simulink model "Regenerative_Braking_Trapezoidal_Control"  (R2023a)
settings: Solver=VariableStepAuto  StartTime=0.0  StopTime=10  RelTol=1e-3
undefined symbols (not defined in the file): Ion, Lithium
libraries: simulink x7, slpidlib x2, spsMeanLib x2, spsPermanentMagnetSynchronousMachineLib x1, spsBatteryLib x1, spsCurrentMeasurementLib x1, spsGroundLib x1, eePwmGenerator x1, spsUniversalBridgeLib x1, spsVoltageMeasurementLib x1, spspowerguiLib x1
settings Model: Creator=Kalyani  LastModifiedBy=hanna
settings DataIOCC: ReturnWorkspaceOutputs=off
settings RTWCC: GPUComputeCapability=5.0
settings ConfigComp: CovBoundaryAbsTol=1.0e-5

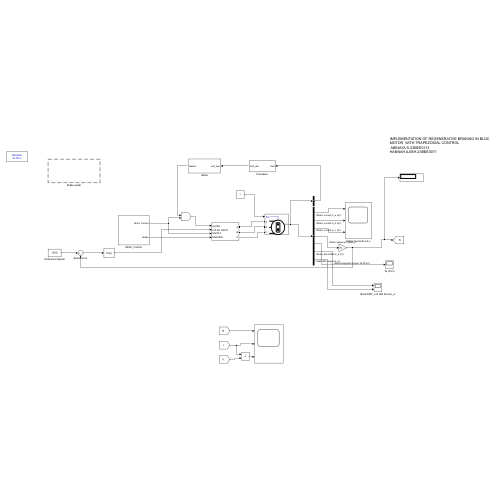
[thumbnail: Simulink's stored preview of the top-level diagram]
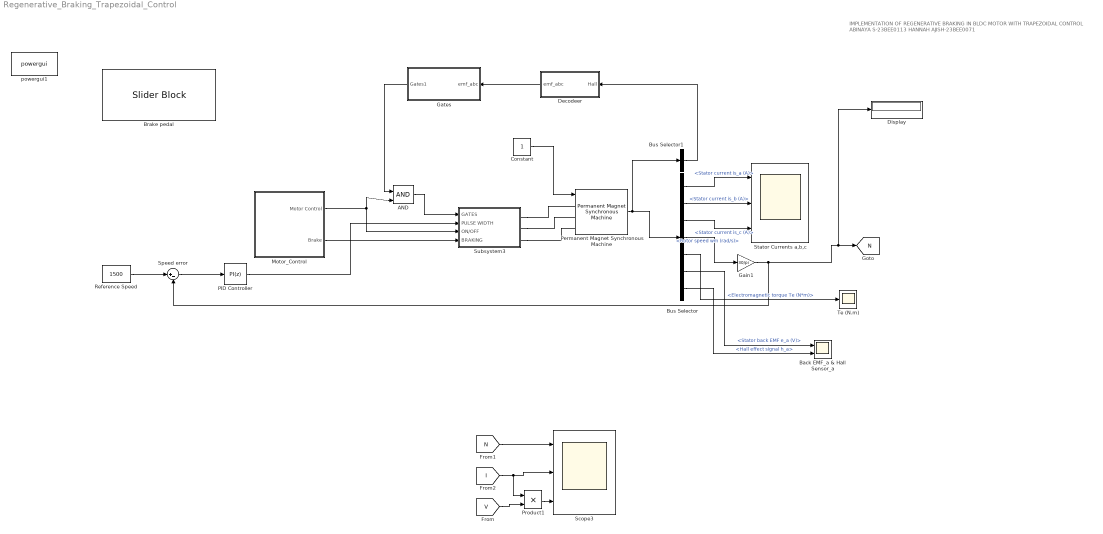
== system Regenerative_Braking_Trapezoidal_Control ==
  note: IMPLEMENTATION OF REGENERATIVE BRAKING IN BLDC MOTOR WITH TRAPEZOIDAL CONTROL
      | ABINAYA S-23BEE0113
      | HANNAH AJISH-23BEE0071
  AND : Logic  IconShape=distinctive  AllPortsSameDT=off  OutDataTypeStr=boolean
  Back EMF_a & Hall Sensor_a : Scope  NumInputPorts=2
  Brake pedal : SliderBlock  ScaleMax=0.949999
  Bus Selector : BusSelector  OutputSignals=Stator current is_a (A),Stator current is_b (A),Stator current is_c (A),Rotor speed wm (rad/s),Electromagnetic torque Te (N*m),Stator back EMF e_a (V),Hall effect signal h_a
  Bus Selector1 : BusSelector  OutputSignals=Hall effect signal h_a,Hall effect signal h_b,Hall effect signal h_c  OutputAsBus=on
  Constant : Constant
  Decodeer : Subsystem
  Display : Display
  Gain1 : Gain  Gain=30/pi
  Gates : Subsystem
  Motor_Control : Subsystem
  PID Controller : slpidlib/PID Controller  Controller=PI  Form=Parallel  TimeDomain=Discrete-time  UseExternalTs=off  SampleTime=-1  IntegratorMethod=Forward Euler  FilterMethod=Forward Euler  ControllerParametersSource=internal  P=0.014  I=0.2288  UseKiTs=off  D=0  N=100  UseFilter=on  TunerSelectOption=Transfer Function Based (PID Tuner App)  InitialConditionSource=internal  InitialConditionForIntegrator=0  InitialConditionForFilter=0  DifferentiatorICPrevScaledInput=0  ExternalReset=none  TrackingMode=off  Kt=1  LimitOutput=off  SatLimitsSource=internal  UpperSaturationLimit=inf  LowerSaturationLimit=-inf  LinearizeAsGain=on  AntiWindupMode=none  Kb=1  LimitIntegrator=off  UpperIntegratorSaturationLimit=inf  LowerIntegratorSaturationLimit=-inf  POutMin=[]  POutMax=[]  IOutMin=[]  IOutMax=[]  DOutMin=[]  DOutMax=[]  NOutMin=[]  NOutMax=[]  SumOutMin=[]  SumOutMax=[]  SaturationOutMin=[]  SaturationOutMax=[]  PParamMin=[]  PParamMax=[]  IParamMin=[]  IParamMax=[]  DParamMin=[]  DParamMax=[]  NParamMin=[]  NParamMax=[]  KbParamMin=[]  KbParamMax=[]  KtParamMin=[]  KtParamMax=[]  KbOutMin=[]  KbOutMax=[]  KtOutMin=[]  KtOutMax=[]  IntegratorOutMin=[]  IntegratorOutMax=[]  FilterOutMin=[]  FilterOutMax=[]  SumI1OutMin=[]  SumI1OutMax=[]  SumI2OutMin=[]  SumI2OutMax=[]  SumI3OutMin=[]  SumI3OutMax=[]  SumI4OutMin=[]  SumI4OutMax=[]  SumDOutMin=[]  SumDOutMax=[]  DifferentiatorOutMin=[]  DifferentiatorOutMax=[]  FilterDiffOutCoefMin=[]  FilterDiffOutCoefMax=[]  ReciprocalOutMin=[]  ReciprocalOutMax=[]  SumDenOutMin=[]  SumDenOutMax=[]  SumNumOutMin=[]  SumNumOutMax=[]  DivideOutMin=[]  DivideOutMax=[]  UdiffTsProdOutMin=[]  UdiffTsProdOutMax=[]  NTsProdOutMin=[]  NTsProdOutMax=[]  UintegralTsProdOutMin=[]  UintegralTsProdOutMax=[]  UngainTsProdOutMin=[]  UngainTsProdOutMax=[]  ClampingZeroOutDataTypeStr=Inherit: Inherit via back propagation  ClampingZeroOutMin=[]  ClampingZeroOutMax=[]  FilterDenConstantOutDataTypeStr=Inherit: Inherit via back propagation  FilterDenConstantOutMin=[]  FilterDenConstantOutMax=[]  PCopyOutDataTypeStr=Inherit: Inherit via back propagation  PCopyOutMin=[]  PCopyOutMax=[]  NCopyOutDataTypeStr=Inherit: Inherit via back propagation  NCopyOutMin=[]  NCopyOutMax=[]  IntegratorContinuousStateAttributes=''  IntegratorStateMustResolveToSignalObject=off  IntegratorRTWStateStorageClass=Auto  FilterContinuousStateAttributes=''  FilterStateMustResolveToSignalObject=off  FilterRTWStateStorageClass=Auto  ParallelPVariant=InternalParameters  IdealPVariant=Disabled  IVariant=InternalParameters  DVariant=Disabled  IntegratorVariant=Discrete  SatVariant=Disabled  AWVariant=Passthrough  PCopyVariant=Disabled  TRVariant=Disabled  FdbkBlocksVariant=Forward  IdealPFdbkVariant=Disabled  SatFdbkVariant=Disabled  DerivativeFilterVariant=Disabled  NVariant=Disabled  NCopyVariant=Disabled_SignalSpec  FilterICVariant=Disabled  IntegratorICVariant=InternalICs  ExternalResetVariant=Disabled  TRSumVariant=Passthrough  SumFdbkVariant=Disabled  SumVariant=Sum_PI  TsampFilterVariant=InternalTs  TsampNgainVariant=Passthrough  TsampIntegralVariant=Disabled_SignalSpec  ExternalSaturationOutDataTypeStr=Inherit: Same as second input
  Permanent Magnet Synchronous Machine : spsPermanentMagnetSynchronousMachineLib/Permanent Magnet Synchronous Machine  NbPhases=3  FluxDistribution=Trapezoidal  RotorType=Round  MechanicalLoad=Torque Tm  PresetModel=No  ShowDetailedParameters=on  MeasurementBus=off  Resistance=0.0095  Inductance=0.0144e-3  dqInductances=[8.5e-3,8.5e-3]  La=0.000395  MachineConstant=Torque Constant (N.m / A_peak)  Flux=0.030794  VoltageCst=51.5954  TorqueCst=0.4927  Flat=120  Mechanical=[0.00019, 1e-6, 8, 0]  PolePairs=4  InitialConditions=[0,0, 0,0]  InitialConditions5ph=[0 0 0 0 0 0]  RefAngle=90 degrees behind phase A axis (modified Park)  IterativeDiscreteModel=Trapezoidal non iterative  TsBlock=-1  TsPowergui=0
  Product1 : Product
  Reference Speed : Constant  Value=1500
  Scope3 : Scope  NumInputPorts=3
  Speed error : Sum  Inputs=|+-
  Stator Currents a,b,c : Scope  NumInputPorts=3
  Subsystem3 : Subsystem
  Te (N.m) : Scope
  powergui1 : spspowerguiLib/powergui  Priority=1  SimulationMode=Discrete  SampleTime=0.00001  frequency=60  Iterations=50  frequencyindice=0  Pbase=100e6  ErrMax=1e-4  UnitsV=kV  UnitsW=MW  buscounter=0  FunctionMessages=off  echomessages=off  EnableUseOfTLC=off  CurrentSourceSwitches=off  DisableSnubberDevices=off  DisableRonSwitches=off  DisableVfSwitches=off  DisplayEquations=off  AutomaticDiscreteSolvers=off  SolverType=Tustin/Backward Euler (TBE)  Interpol=off  ExternalGateDelay=off  methode=off  Ts=100  x0status=blocks  SPID=on  SwTol=0  HookPort=off  NonlinearTolerance=1e-4  nMaxIteration=100  ContinueOnMaxIteration=off  RestoreLinks=warning  ResistiveCurrentMeasurement=off  Frange=[0:2:500]  Ylog=off  Xlog=on  ShowGrid=off  save=off  variable=ZData  structure=0  ZoomFFT=off  StartTime=0.0  cycles=1  DisplayStyle=1  fundamental=60  FreqAxis=off  MaxFrequency=1000  frequencyindicesteady=1  RmsSteady=1  display=off
  tag scope: N=global
  wires:
  [N] -> Scope3/1
  Product1/1 -> Scope3/3
  Bus Selector/1 -> Stator Currents a,b,c/1  "<Stator current is_a (A)>"
  Bus Selector/2 -> Stator Currents a,b,c/2  "<Stator current is_b (A)>"
  Bus Selector/3 -> Stator Currents a,b,c/3  "<Stator current is_c (A)>"
  Bus Selector/4 -> Gain1/1  "<Rotor speed wm (rad/s)>"
  Bus Selector/5 -> Te (N.m)/1  "<Electromagnetic torque Te (N*m)>"
  Bus Selector/6 -> Back EMF_a & Hall Sensor_a/1  "<Stator back EMF e_a (V)>"
  Bus Selector/7 -> Back EMF_a & Hall Sensor_a/2  "<Hall effect signal h_a>"
  Permanent Magnet Synchronous Machine/1 -> Bus Selector1/1, Bus Selector/1
  Reference Speed/1 -> Speed error/1
  Speed error/1 -> PID Controller/1
  Decodeer/1(emf_abc) -> Gates/1(emf_abc)
  [V] -> Product1/2
  [I] -> Product1/1, Scope3/2
  Motor_Control/2(Brake) -> Subsystem3/4(BRAKING)
  Motor_Control/1(Motor Control) -> AND/2, Subsystem3/3(ON/OFF)
  Gates/1(Gates1) -> AND/1
  AND/1 -> Subsystem3/1(GATES)
  Gain1/1 -> Speed error/2, Display/1, [N]
  PID Controller/1 -> Subsystem3/2(PULSE WIDTH)
  Bus Selector1/1 -> Decodeer/1(Hall)
  Constant/1 -> Permanent Magnet Synchronous Machine/1
  connections:
  Subsystem3/RConn2 -- Permanent Magnet Synchronous Machine/LConn2
  Subsystem3/RConn3 -- Permanent Magnet Synchronous Machine/LConn3
  Subsystem3/RConn1 -- Permanent Magnet Synchronous Machine/LConn1

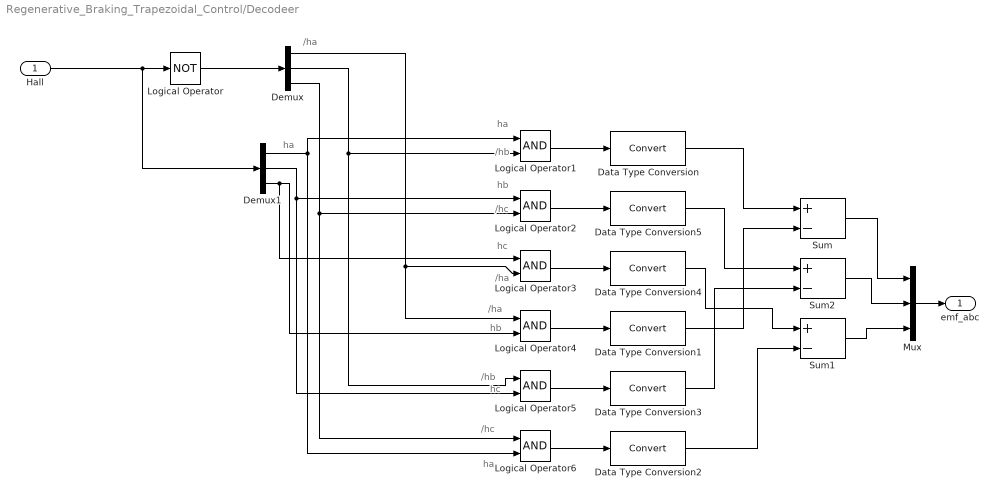
== system Regenerative_Braking_Trapezoidal_Control/Decodeer ==
  note: ha
  note: /ha
  note: /hb
  note: /hc
  note: /ha
  note: /ha
  note: /hb
  note: /hc
  note: ha
  note: hb
  note: hc
  note: hb
  note: hc
  note: ha
  Hall : Inport
  Data Type Conversion{,1..5} (6 alike) : DataTypeConversion  SaturateOnIntegerOverflow=off  RndMeth=Floor
  Demux : Demux  Outputs=3
  Demux1 : Demux  Outputs=3
  Logical Operator : Logic  Operator=NOT  AllPortsSameDT=off  OutDataTypeStr=boolean
  Logical Operator{1..6} (6 alike) : Logic  AllPortsSameDT=off  OutDataTypeStr=boolean
  Mux : Mux  Inputs=3
  Sum : Sum  Inputs=+-
  Sum1 : Sum  Inputs=+-
  Sum2 : Sum  Inputs=+-
  emf_abc : Outport
  wires:
  Logical Operator/1 -> Demux/1
  Demux/1 -> Logical Operator4/1, Logical Operator3/2
  Demux/2 -> Logical Operator5/1, Logical Operator1/2
  Demux/3 -> Logical Operator6/1, Logical Operator2/2
  Demux1/1 -> Logical Operator6/2, Logical Operator1/1
  Demux1/2 -> Logical Operator5/2, Logical Operator2/1
  Demux1/3 -> Logical Operator3/1, Logical Operator4/2
  Logical Operator1/1 -> Data Type Conversion/1
  Logical Operator2/1 -> Data Type Conversion5/1
  Logical Operator3/1 -> Data Type Conversion4/1
  Logical Operator4/1 -> Data Type Conversion1/1
  Logical Operator5/1 -> Data Type Conversion3/1
  Logical Operator6/1 -> Data Type Conversion2/1
  Data Type Conversion/1 -> Sum/1
  Data Type Conversion1/1 -> Sum/2
  Data Type Conversion5/1 -> Sum2/1
  Data Type Conversion3/1 -> Sum2/2
  Data Type Conversion2/1 -> Sum1/2
  Data Type Conversion4/1 -> Sum1/1
  Sum/1 -> Mux/1
  Sum2/1 -> Mux/2
  Sum1/1 -> Mux/3
  Mux/1 -> emf_abc/1
  Hall/1 -> Demux1/1, Logical Operator/1

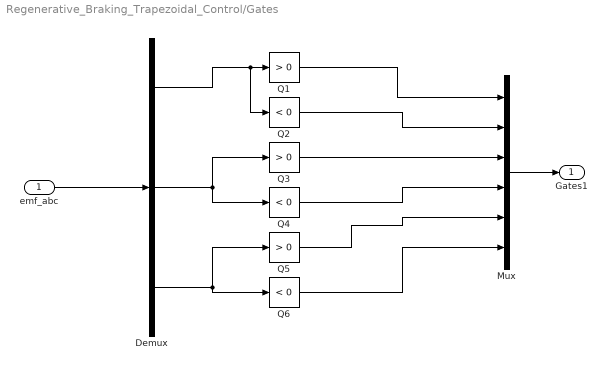
== system Regenerative_Braking_Trapezoidal_Control/Gates ==
  emf_abc : Inport
  Demux : Demux  Outputs=3
  Mux : Mux  Inputs=6
  Q1 : simulink/Logic and Bit Operations/Compare To Constant  relop=>  const=0  OutDataTypeStr=boolean
  Q2 : simulink/Logic and Bit Operations/Compare To Constant  relop=<  const=0  OutDataTypeStr=boolean
  Q3 : simulink/Logic and Bit Operations/Compare To Constant  relop=>  const=0  OutDataTypeStr=boolean
  Q4 : simulink/Logic and Bit Operations/Compare To Constant  relop=<  const=0  OutDataTypeStr=boolean
  Q5 : simulink/Logic and Bit Operations/Compare To Constant  relop=>  const=0  OutDataTypeStr=boolean
  Q6 : simulink/Logic and Bit Operations/Compare To Constant  relop=<  const=0  OutDataTypeStr=boolean
  Gates1 : Outport
  wires:
  emf_abc/1 -> Demux/1
  Mux/1 -> Gates1/1
  Demux/1 -> Q2/1, Q1/1
  Demux/3 -> Q5/1, Q6/1
  Demux/2 -> Q3/1, Q4/1
  Q1/1 -> Mux/1
  Q2/1 -> Mux/2
  Q3/1 -> Mux/3
  Q4/1 -> Mux/4
  Q5/1 -> Mux/5
  Q6/1 -> Mux/6

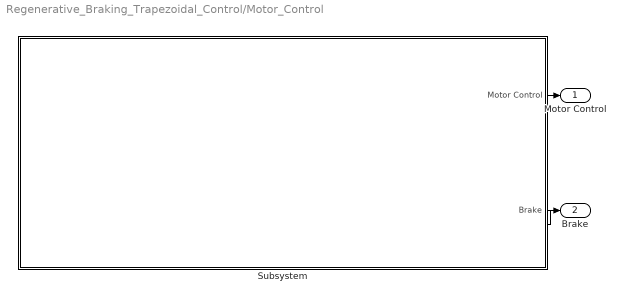
== system Regenerative_Braking_Trapezoidal_Control/Motor_Control ==
  Subsystem : Subsystem
  Motor Control : Outport
  Brake : Outport  Port=2
  wires:
  Subsystem/1(Motor Control) -> Motor Control/1
  Subsystem/2(Brake) -> Brake/1

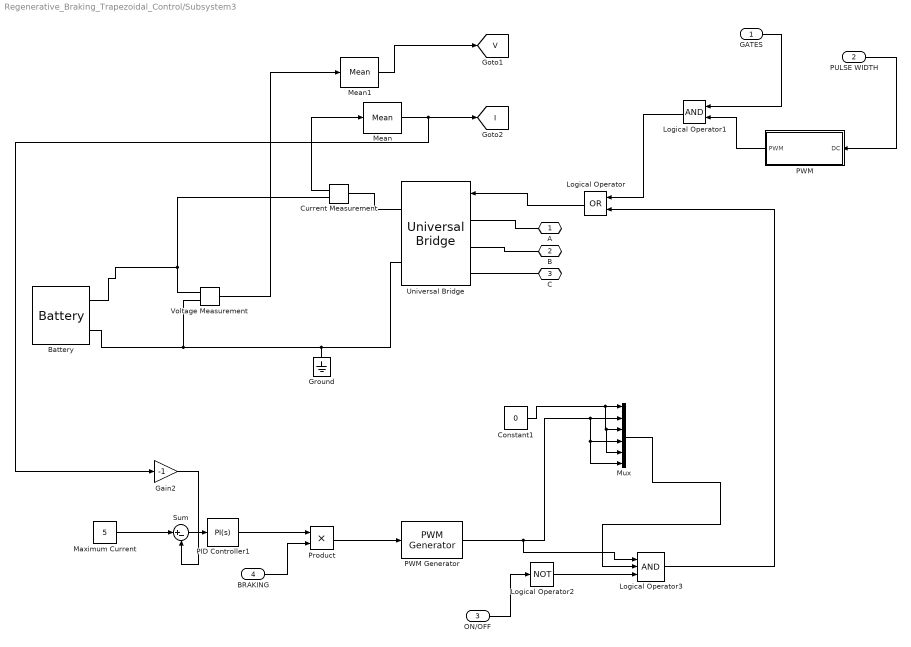
== system Regenerative_Braking_Trapezoidal_Control/Subsystem3 ==
  GATES : Inport
  PULSE WIDTH : Inport  Port=2
  ON/OFF : Inport  Port=3
  BRAKING : Inport  Port=4
  Battery : spsBatteryLib/Battery  BatType=Lithium-Ion  NomV=300  NomQ=50  SOC=50  Batt_Tr=30  PresetModel=on  MaxQ=50  MinV=225  FullV=349.1961  Dis_rate=21.7391  R=0.06  Normal_OP=45.2174  expZone="[324.1158      2.456522]"
  Constant1 : Constant  Value=0
  Current Measurement : spsCurrentMeasurementLib/Current Measurement  PhasorSimulation=off  OutputType=Complex  PSBequivalent=0
  Gain2 : Gain  Gain=-1
  Ground : spsGroundLib/Ground  LConnTagsString=a
  Logical Operator : Logic  Operator=OR  AllPortsSameDT=off  OutDataTypeStr=boolean
  Logical Operator1 : Logic  AllPortsSameDT=off  OutDataTypeStr=boolean
  Logical Operator2 : Logic  Operator=NOT  AllPortsSameDT=off  OutDataTypeStr=boolean
  Logical Operator3 : Logic  Inputs=3  AllPortsSameDT=off  OutDataTypeStr=boolean
  Maximum Current : Constant  Value=5
  Mean : spsMeanLib/Mean  Freq=60  Vinit=0  Ts=0
  Mean1 : spsMeanLib/Mean  Freq=60  Vinit=0  Ts=0
  Mux : Mux  Inputs=6
  PID Controller1 : slpidlib/PID Controller  Controller=PI  Form=Parallel  TimeDomain=Continuous-time  UseExternalTs=off  SampleTime=-1  IntegratorMethod=Forward Euler  FilterMethod=Forward Euler  ControllerParametersSource=internal  P=1  I=25  UseKiTs=off  D=0  N=100  UseFilter=on  TunerSelectOption=Transfer Function Based (PID Tuner App)  InitialConditionSource=internal  InitialConditionForIntegrator=0  InitialConditionForFilter=0  DifferentiatorICPrevScaledInput=0  ExternalReset=none  TrackingMode=off  Kt=1  LimitOutput=off  SatLimitsSource=internal  UpperSaturationLimit=10  LowerSaturationLimit=-10  LinearizeAsGain=on  AntiWindupMode=back-calculation  Kb=0.01665  LimitIntegrator=off  UpperIntegratorSaturationLimit=inf  LowerIntegratorSaturationLimit=-inf  POutMin=[]  POutMax=[]  IOutMin=[]  IOutMax=[]  DOutMin=[]  DOutMax=[]  NOutMin=[]  NOutMax=[]  SumOutMin=[]  SumOutMax=[]  SaturationOutMin=[]  SaturationOutMax=[]  PParamMin=[]  PParamMax=[]  IParamMin=[]  IParamMax=[]  DParamMin=[]  DParamMax=[]  NParamMin=[]  NParamMax=[]  KbParamMin=[]  KbParamMax=[]  KtParamMin=[]  KtParamMax=[]  KbOutMin=[]  KbOutMax=[]  KtOutMin=[]  KtOutMax=[]  IntegratorOutMin=[]  IntegratorOutMax=[]  FilterOutMin=[]  FilterOutMax=[]  SumI1OutMin=[]  SumI1OutMax=[]  SumI2OutMin=[]  SumI2OutMax=[]  SumI3OutMin=[]  SumI3OutMax=[]  SumI4OutMin=[]  SumI4OutMax=[]  SumDOutMin=[]  SumDOutMax=[]  DifferentiatorOutMin=[]  DifferentiatorOutMax=[]  FilterDiffOutCoefMin=[]  FilterDiffOutCoefMax=[]  ReciprocalOutMin=[]  ReciprocalOutMax=[]  SumDenOutMin=[]  SumDenOutMax=[]  SumNumOutMin=[]  SumNumOutMax=[]  DivideOutMin=[]  DivideOutMax=[]  UdiffTsProdOutMin=[]  UdiffTsProdOutMax=[]  NTsProdOutMin=[]  NTsProdOutMax=[]  UintegralTsProdOutMin=[]  UintegralTsProdOutMax=[]  UngainTsProdOutMin=[]  UngainTsProdOutMax=[]  ClampingZeroOutDataTypeStr=Inherit: Inherit via back propagation  ClampingZeroOutMin=[]  ClampingZeroOutMax=[]  FilterDenConstantOutDataTypeStr=Inherit: Inherit via back propagation  FilterDenConstantOutMin=[]  FilterDenConstantOutMax=[]  PCopyOutDataTypeStr=Inherit: Inherit via back propagation  PCopyOutMin=[]  PCopyOutMax=[]  NCopyOutDataTypeStr=Inherit: Inherit via back propagation  NCopyOutMin=[]  NCopyOutMax=[]  IntegratorContinuousStateAttributes=''  IntegratorStateMustResolveToSignalObject=off  IntegratorRTWStateStorageClass=Auto  FilterContinuousStateAttributes=''  FilterStateMustResolveToSignalObject=off  FilterRTWStateStorageClass=Auto  ParallelPVariant=InternalParameters  IdealPVariant=Disabled  IVariant=InternalParameters  DVariant=Disabled  IntegratorVariant=Continuous  SatVariant=Disabled  AWVariant=Passthrough  PCopyVariant=Disabled  TRVariant=Disabled  FdbkBlocksVariant=Forward  IdealPFdbkVariant=Disabled  SatFdbkVariant=Disabled  DerivativeFilterVariant=Disabled  NVariant=Disabled  NCopyVariant=Disabled_SignalSpec  FilterICVariant=Disabled  IntegratorICVariant=InternalICs  ExternalResetVariant=Disabled  TRSumVariant=Passthrough  SumFdbkVariant=Disabled  SumVariant=Sum_PI  TsampFilterVariant=InternalTs  TsampNgainVariant=Passthrough  TsampIntegralVariant=Disabled_SignalSpec  ExternalSaturationOutDataTypeStr=Inherit: Same as second input
  PWM : Subsystem
  PWM Generator : eePwmGenerator/PWM Generator  CarrCount=Up  Tper=5e-04  Tdelay=0  Ts=0.00001
  Product : Product
  Sum : Sum  Inputs=|+-
  Universal Bridge : spsUniversalBridgeLib/Universal Bridge  Arms=3  SnubberResistance=1e5  SnubberCapacitance=inf  Device=IGBT / Diodes  Ron=1e-3  Lon=0  ForwardVoltages="[  0  0  ]"  ForwardVoltage=0  GTOparameters=[ 10e-6 , 20e-6 ]  IGBTparameters=[ 1e-6 , 2e-6 ]  Measurements=None  Measurements_2=None  converterType=Rectifier
  Voltage Measurement : spsVoltageMeasurementLib/Voltage Measurement  PhasorSimulation=off  OutputType=Complex  PSBequivalent=0
  A : PMIOPort  Side=Right
  B : PMIOPort  Port=2  Side=Right
  C : PMIOPort  Port=3  Side=Right
  tag scope: I=global, V=global
  wires:
  Logical Operator2/1 -> Logical Operator3/3
  Voltage Measurement/1 -> Mean1/1
  Sum/1 -> PID Controller1/1
  Product/1 -> PWM Generator/1
  Constant1/1 -> Mux/5, Mux/3, Mux/1
  Maximum Current/1 -> Sum/1
  Current Measurement/1 -> Mean/1
  Logical Operator3/1 -> Logical Operator/2
  Mux/1 -> Logical Operator3/2
  Gain2/1 -> Sum/2
  Logical Operator1/1 -> Logical Operator/1
  PWM/1(PWM) -> Logical Operator1/2
  PULSE WIDTH/1 -> PWM/1(DC)
  GATES/1 -> Logical Operator1/1
  PWM Generator/1 -> Logical Operator3/1, Mux/4, Mux/6, Mux/2
  Logical Operator/1 -> Universal Bridge/1
  Mean/1 -> Gain2/1, [I]
  Mean1/1 -> [V]
  BRAKING/1 -> Product/2
  ON/OFF/1 -> Logical Operator2/1
  PID Controller1/1 -> Product/1
  connections:
  Voltage Measurement/LConn1 -- Current Measurement/RConn1 -- Battery/LConn1
  Voltage Measurement/LConn2 -- Ground/LConn1 -- Universal Bridge/RConn2 -- Battery/LConn2
  Universal Bridge/RConn1 -- Current Measurement/LConn1
  A/RConn1 -- Universal Bridge/LConn1
  Universal Bridge/LConn2 -- B/RConn1
  C/RConn1 -- Universal Bridge/LConn3

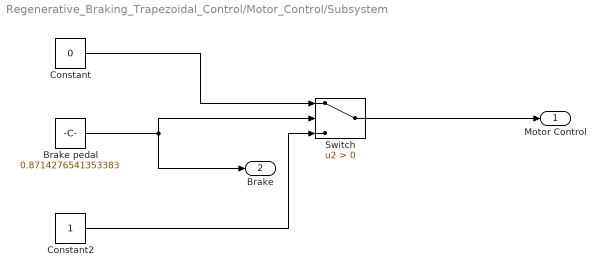
== system Regenerative_Braking_Trapezoidal_Control/Motor_Control/Subsystem ==
  Brake pedal : Constant  Value=0.8714276541353383
  Constant : Constant  Value=0
  Constant2 : Constant
  Switch : Switch  Criteria=u2 > Threshold  SaturateOnIntegerOverflow=off  InputSameDT=off
  Motor Control : Outport
  Brake : Outport  Port=2
  wires:
  Switch/1 -> Motor Control/1
  Constant/1 -> Switch/1
  Brake pedal/1 -> Brake/1, Switch/2
  Constant2/1 -> Switch/3

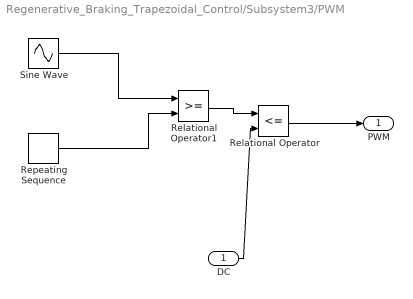
== system Regenerative_Braking_Trapezoidal_Control/Subsystem3/PWM ==
  DC : Inport
  Relational Operator : RelationalOperator  Operator=<=  OutDataTypeStr=boolean  RndMeth=Simplest  InputSameDT=off
  Relational Operator1 : RelationalOperator  OutDataTypeStr=boolean  RndMeth=Simplest  InputSameDT=off
  Repeating Sequence : simulink/Sources/Repeating Sequence  rep_seq_t=[0 2]  rep_seq_y=[0 2]
  Sine Wave : Sin  SampleTime=0
  PWM : Outport
  wires:
  Sine Wave/1 -> Relational Operator1/1
  Repeating Sequence/1 -> Relational Operator1/2
  Relational Operator1/1 -> Relational Operator/1
  Relational Operator/1 -> PWM/1
  DC/1 -> Relational Operator/2
